simulink model "KinarmFlankerTask_260119"  (R2019b)
settings: Solver=ode4  StartTime=0.0  StopTime=inf  FixedStep=BKIN_STEP_TIME  RelTol=1e-3  EnableMultiTasking=on
StartFcn:
  |  warndlg('Dexterit-E models cannot run under simulation. Please compile your model and run it from within Dexterit-E.');set_param(bdroot,'SimulationCommand','stop')
model workspace (MAT data in the model file):
  ANT_ON = 7
  BKIN_KINEMATIC_FRAME_SIZE = 400
  BKIN_STEP_TIME = 0.00025
  CENTRE_TARG_COL = 8
  CUE_DELAY = 12
  CUE_ON_TIME = 11
  CUE_RAND = 13
  CUE_TARG_COL = 9
  DISTRACT_TARG_COL = 7
  E_ARROWS_BOT = 19
  E_ARROWS_OFF = 23
  E_ARROWS_ON = 21
  E_ARROWS_TOP = 18
  E_CENTRE_LEFT = 14
  E_CENTRE_RIGHT = 15
  E_CONG = 16
  E_CORRECT = 22
  E_CUE_BOT = 7
  E_CUE_BOTH = 8
  E_CUE_CENT = 20
  E_CUE_NONE = 5
  E_CUE_OFF = 9
  E_CUE_TOP = 6
  E_DISTRACT_LEFT = 11
  E_DISTRACT_NEUT = 13
  E_DISTRACT_RIGHT = 12
  E_FALSE_START = 28
  E_INCONG = 17
  E_INCORRECT = 24
  E_LEFT_REACHED = 1
  E_NEUTRAL = 10
  E_NO_EVENT = 0
  E_RIGHT_REACHED = 2
  E_TIMED_OUT = 29
  E_TRIAL_END = 30
  E_TRIAL_START = 3
  E_WALLS_ON = 4
  FLICKER_ON = 9
  FLICKER_TIME = 10
  IMAGE_1 = 6
  IMAGE_2 = 7
  IMAGE_3 = 8
  LBARR_TARG_COL = 4
  LENGTH = 3
  LOAD_X = 1
  LOAD_Y = 2
  LWALL_TARG_COL = 3
  NEUT_ON = 8
  PERTURB_SET = 10
  POSTRESP_DELAY = 4
  RADIUS_VIS = 3
  RBARR_TARG_COL = 6
  REACH_DELAY = 1
  REACH_RAND = 2
  REACH_TO = 3
  RESULT_TARG_COL = 2
  RWALL_TARG_COL = 5
  SPRING_CONST = 5
  START_TARG_COL = 1
  STROKE_WIDTH = 11
  TARG_LENGTH = 3
  TARG_WIDTH = 4
  TEXT = 9
  TEXT_SIZE = 10
  WALL_SHAKE_TOGGLE = 6
  WIDTH = 4
  Width = 4
  X_LENGTH = 4
  Y_LENGTH = 5
  col_x = 1
  col_y = 2
undefined symbols (not defined in the file or in its folder): slselsubs
libraries: Video x10, General x3, KINARM_general x3, KINARM_EP_loads x2
settings Model: ModifiedComment=chris -- Wed Feb 16 09:18:30 2005 -- Version 1.1384  ModifiedHistory=Feb 16/05 - Add error repeat, add offset ramp  ExtModeArmWhenConnect=off  ExtModeLogAll=off  OrderedModelArguments=off  Creator=Chris Grebeldinger  LastModifiedBy=apark2
settings SolverCC: AutoInsertRateTranBlk=on
settings DataIOCC: SaveFormat=Array  SignalLoggingSaveFormat=ModelDataLogs  SaveOutput=off  SaveTime=off  ReturnWorkspaceOutputs=off  SignalLoggingName=sigsOut
settings OptimizationCC: BlockReduction=off  BooleanDataType=off  OptimizeBlockIOStorage=off  BufferReuse=off  GlobalBufferReuse=off  ExpressionFolding=off  ExpressionDepthLimit=2147483647  LocalBlockOutputs=off  InitFltsAndDblsToZero=on  LifeSpan=inf  OptimizeDataStoreBuffers=off  BusAssignmentInplaceUpdate=off
settings DebuggingCC: SaveWithParameterizedLinksMsg=none  UnderspecifiedInitializationDetection=Classic  MergeDetectMultiDrivingBlocksExec=none  SignalResolutionControl=TryResolveAllWithWarning  MultiTaskDSMMsg=warning  FcnCallInpInsideContextMsg=warning  BusObjectLabelMismatch=none  StateNameClashWarn=warning  StrictBusMsg=ErrorOnBusTreatedAsVector  SFUnexpectedBacktrackingDiag=warning  SFNoUnconditionalDefaultTransitionDiag=warning  SFExecutionAtInitializationDiag=none  ArithmeticOperatorsInVariantConditions=warning
settings HardwareCC: ProdBitPerPointer=32  ProdBitPerSizeT=32  ProdBitPerPtrDiffT=32  ProdLargestAtomicFloat=None  ProdWordSize=32  ProdLongLongMode=on  ProdHWDeviceType=Generic->32-bit x86 compatible  TargetLongLongMode=on  TargetIntDivRoundTo=Zero  TargetEndianess=LittleEndian  TargetHWDeviceType=Generic->32-bit x86 compatible
settings ModelReferenceCC: PropagateSignalLabelsOutOfModel=off
settings SFSimCC: SimCustomHeaderCode="#include \"stdlib.h\""  SimUseLocalCustomCode=off  SimParseCustomCode=off  CustomCodeUndefinedFunction=UseInterfaceOnly
settings RTWCC: Description=Simulink Real-Time  SystemTargetFile=slrt.tlc  TemplateMakefile=slrt_default_tmf  RTWUseLocalCustomCode=off  CustomSourceCode="#include \"stdlib.h\""  CodeExecutionProfiling=on
settings CodeAppCC: MaxIdLength=63  StateflowObjectComments=on
settings SimulinkRealTimeCC: TargetFcnLib=ansi_tfl_tmw.mat  GeneratePreprocessorConditionals=Disable all  PreserveStateflowLocalDataDimensions=off
settings ConfigComp: CovMetricSettings=dw  CovHtmlReporting=on  CovSaveCumulativeToWorkspaceVar=on  CovSaveSingleToWorkspaceVar=on  CovExternalEMLEnable=off

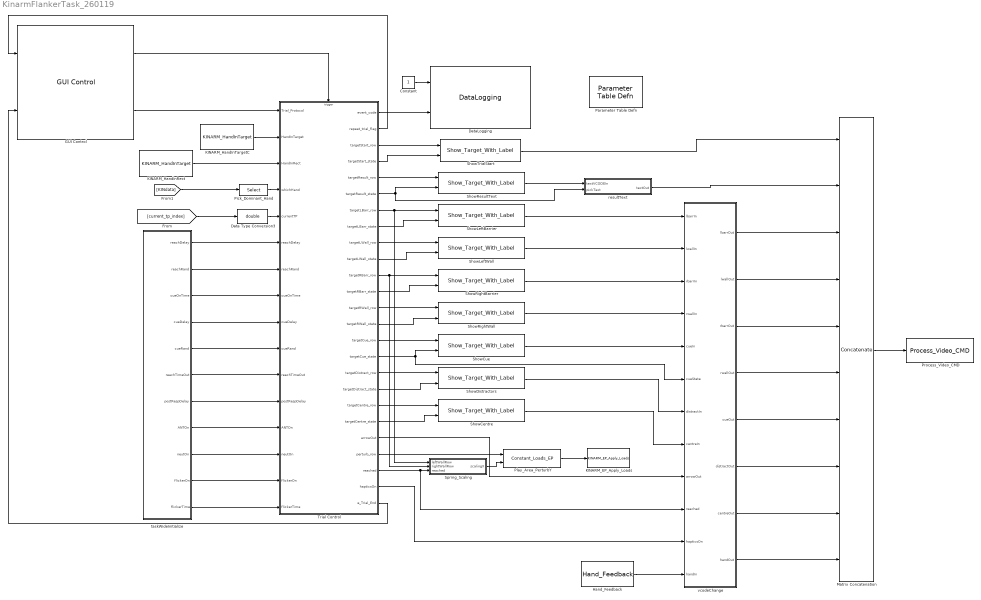
== system KinarmFlankerTask_260119 ==
  Constant : Constant
  Data Type Conversion3 : DataTypeConversion  OutDataTypeStr=double
  DataLogging : General/DataLogging  log_event_codes=on  log_analog_inputs=off  show_time_remaining=off  ecat_include=on
  GUI Control : General/GUI Control  task_version=1.0  show_repeat_trial_flag=on  use_custom_tp=off  target_type_str=Circle  Target_Type=1  XYcols=[1 2]  Vcols=3  Lcols=4  indices_padding=[0 0 0 0;0 0 0 0]  target_table_rows=64  load_table_rows=20  tp_table_rows=100
  Hand_Feedback : KINARM_general/Hand_Feedback  feedback_cntl_src=none
  KINARM_EP_Apply_Loads : KINARM_EP_loads/KINARM_EP_Apply_Loads  up_duration=1500  down_duration=1500  max_force=20
  KINARM_HandInRect : KINARM_general/KINARM_HandInTarget  use_dominant_hand=on  target_type=Rectangle  num_states=1  attribcol1=[X_LENGTH Y_LENGTH 0]  attribcol2=[0 0 0]  attribcol3=[0 0 0]  attribcol4=[0 0 0]  attribcol5=[0 0 0]
  KINARM_HandInTargetC : KINARM_general/KINARM_HandInTarget  use_dominant_hand=on  target_type=Circle  num_states=1  attribcol1=[RADIUS_VIS]  attribcol2=[0]  attribcol3=[0]  attribcol4=[0]  attribcol5=[0]
  Matrix Concatenation : Concatenate  NumInputs=10  Mode=Multidimensional array
  Parameter Table Defn : General/Parameter Table Defn  ShowInLibBrowser=0
  Pick_Dominant_Hand : Selector  NumberOfDimensions=2  InputPortWidth=3  IndexOptions=Index vector (dialog),Index vector (dialog)  Indices=[3],[1]  OutputSizes=slselsubs([(-2),(-2)],1),slselsubs([(-2),(-2)],2)
  Play_Area_PerturbY : KINARM_EP_loads/Constant_Loads_EP  use_dom_hand=on  loadcol=[LOAD_X LOAD_Y]  source=port  scaling=1  use_LH_coord=on
  Process_Video_CMD : Video/Process_Video_CMD  video_delay=50
  ShowCentre : Video/Show_Target_With_Label  target_type=Rectangle  num_states=2  attribcol1=[IMAGE_1 0 0 X_LENGTH Y_LENGTH 0 0 0 0]  attribcol2=[IMAGE_2 0 0 X_LENGTH Y_LENGTH 0 0 0 0]  attribcol3=[0 0 0 0 0 0 0 0 0]  attribcol4=[0 0 0 0 0 0 0 0 0]  attribcol5=[0 0 0 0 0 0 0 0 0]  stateindices_padding=[0 0;0 0;0 0;0 0;0 0]  source=dialog  opacity=100  target_display=Both subject and operator displays
  ShowCue : Video/Show_Target_With_Label  target_type=Rectangle  num_states=4  attribcol1=[0 0 0 0 0 0 TEXT IMAGE_1 TEXT_SIZE]  attribcol2=[0 0 0 0 0 0 TEXT IMAGE_1 TEXT_SIZE]  attribcol3=[0 0 0 0 0 0 TEXT IMAGE_1 TEXT_SIZE]  attribcol4=[0 0 0 0 0 0 TEXT IMAGE_1 TEXT_SIZE]  attribcol5=[0 0 0 0 0 0 0 0 0]  stateindices_padding=[0 0;0 0;0 0;0 0;0 0]  source=dialog  opacity=100  target_display=Both subject and operator displays
  ShowDistractors : Video/Show_Target_With_Label  target_type=Rectangle  num_states=3  attribcol1=[IMAGE_1 0 0 X_LENGTH Y_LENGTH 0 0 0 0]  attribcol2=[IMAGE_2 0 0 X_LENGTH Y_LENGTH 0 0 0 0]  attribcol3=[IMAGE_3 0 0 X_LENGTH Y_LENGTH 0 0 0 0]  attribcol4=[0 0 0 0 0 0 0 0 0]  attribcol5=[0 0 0 0 0 0 0 0 0]  stateindices_padding=[0 0;0 0;0 0;0 0;0 0]  source=dialog  opacity=100  target_display=Both subject and operator displays
  ShowLeftBarrier : Video/Show_Target_With_Label  target_type=Rectangle  num_states=1  attribcol1=[IMAGE_1 0 0 X_LENGTH Y_LENGTH 0 0 0 0]  attribcol2=[0 0 0 0 0 0 0 0 0]  attribcol3=[0 0 0 0 0 0 0 0 0]  attribcol4=[0 0 0 0 0 0 0 0 0]  attribcol5=[0 0 0 0 0 0 0 0 0]  stateindices_padding=[0 0;0 0;0 0;0 0;0 0]  source=dialog  opacity=100  target_display=Both subject and operator displays
  ShowLeftWall : Video/Show_Target_With_Label  target_type=Rectangle  num_states=2  attribcol1=[IMAGE_1 0 0 X_LENGTH Y_LENGTH 0 0 0 0]  attribcol2=[IMAGE_1 0 0 X_LENGTH Y_LENGTH 0 0 0 0]  attribcol3=[0 0 0 0 0 0 0 0 0]  attribcol4=[0 0 0 0 0 0 0 0 0]  attribcol5=[0 0 0 0 0 0 0 0 0]  stateindices_padding=[0 0;0 0;0 0;0 0;0 0]  source=dialog  opacity=100  target_display=Both subject and operator displays
  ShowResultText : Video/Show_Target_With_Label  target_type=Circle  num_states=4  attribcol1=[0 0 0 0 TEXT IMAGE_2 TEXT_SIZE]  attribcol2=[0 0 0 0 TEXT IMAGE_1 TEXT_SIZE]  attribcol3=[0 0 0 0 TEXT IMAGE_1 TEXT_SIZE]  attribcol4=[0 0 0 0 TEXT IMAGE_1 TEXT_SIZE]  attribcol5=[0 0 0 0 0 0 0]  stateindices_padding=[0 0 0 0;0 0 0 0;0 0 0 0;0 0 0 0;0 0 0 0]  source=dialog  opacity=100  target_display=Both subject and operator displays
  ShowRightBarrier : Video/Show_Target_With_Label  target_type=Rectangle  num_states=1  attribcol1=[IMAGE_1 0 0 X_LENGTH Y_LENGTH 0 0 0 0]  attribcol2=[0 0 0 0 0 0 0 0 0]  attribcol3=[0 0 0 0 0 0 0 0 0]  attribcol4=[0 0 0 0 0 0 0 0 0]  attribcol5=[0 0 0 0 0 0 0 0 0]  stateindices_padding=[0 0;0 0;0 0;0 0;0 0]  source=dialog  opacity=100  target_display=Both subject and operator displays
  ShowRightWall : Video/Show_Target_With_Label  target_type=Rectangle  num_states=2  attribcol1=[IMAGE_1 0 0 X_LENGTH Y_LENGTH 0 0 0 0]  attribcol2=[IMAGE_2 0 0 X_LENGTH Y_LENGTH 0 0 0 0]  attribcol3=[0 0 0 0 0 0 0 0 0]  attribcol4=[0 0 0 0 0 0 0 0 0]  attribcol5=[0 0 0 0 0 0 0 0 0]  stateindices_padding=[0 0;0 0;0 0;0 0;0 0]  source=dialog  opacity=100  target_display=Both subject and operator displays
  ShowTrialStart : Video/Show_Target_With_Label  target_type=Circle  num_states=1  attribcol1=[IMAGE_1 IMAGE_2 STROKE_WIDTH RADIUS_VIS 0 0 0]  attribcol2=[0 0 0 0 0 0 0]  attribcol3=[0 0 0 0 0 0 0]  attribcol4=[0 0 0 0 0 0 0]  attribcol5=[0 0 0 0 0 0 0]  stateindices_padding=[0 0 0 0;0 0 0 0;0 0 0 0;0 0 0 0;0 0 0 0]  source=dialog  opacity=100  target_display=Both subject and operator displays
  Spring_Scaling : Subsystem
  Trial Control : Stateflow chart  TreatAsAtomicUnit=on
  resultText : Subsystem
  taskWideInitialize : Subsystem
  vcodeChange : Subsystem
  wires:
  Trial Control/25(e_Trial_End) -> GUI Control/2
  Matrix Concatenation/1 -> Process_Video_CMD/1
  Trial Control/1(event_code) -> DataLogging/2
  Constant/1 -> DataLogging/1
  GUI Control/2 -> Trial Control/1(Trial_Protocol)
  Trial Control/2(repeat_trial_flag) -> GUI Control/1
  [current_tp_index] -> Data Type Conversion3/1
  ShowResultText/1 -> resultText/1(textVCODEIn)
  KINARM_HandInTargetC/1 -> Trial Control/2(HandInTarget)
  GUI Control/1 -> Trial Control/Trigger
  Data Type Conversion3/1 -> Trial Control/5(currentTP)
  Trial Control/18(targetDistract_state) -> ShowDistractors/2
  Trial Control/17(targetDistract_row) -> ShowDistractors/1
  Trial Control/13(targetRWall_row) -> ShowRightWall/1
  Trial Control/9(targetLWall_row) -> ShowLeftWall/1
  Trial Control/10(targetLWall_state) -> ShowLeftWall/2
  Trial Control/5(targetResult_row) -> ShowResultText/1
  Trial Control/6(targetResult_state) -> resultText/2(pickText), ShowResultText/2
  Trial Control/19(targetCentre_row) -> ShowCentre/1
  Trial Control/20(targetCentre_state) -> ShowCentre/2
  taskWideInitialize/1(reachDelay) -> Trial Control/6(reachDelay)
  taskWideInitialize/7(postRespDelay) -> Trial Control/12(postRespDelay)
  Trial Control/14(targetRWall_state) -> ShowRightWall/2
  resultText/1(textOut) -> Matrix Concatenation/2
  Play_Area_PerturbY/1 -> KINARM_EP_Apply_Loads/1
  Trial Control/24(hapticsOn) -> vcodeChange/11(hapticsOn)
  Trial Control/22(perturb_row) -> Play_Area_PerturbY/1
  Trial Control/3(targetStart_row) -> ShowTrialStart/1
  Trial Control/4(targetStart_state) -> ShowTrialStart/2
  ShowTrialStart/1 -> Matrix Concatenation/1
  taskWideInitialize/6(reachTimeOut) -> Trial Control/11(reachTimeOut)
  Trial Control/23(reached) -> Spring_Scaling/3(reached), vcodeChange/10(reached)
  ShowLeftWall/1 -> vcodeChange/2(lwallIn)
  ShowRightWall/1 -> vcodeChange/4(rwallIn)
  vcodeChange/6("distractOut ") -> Matrix Concatenation/8
  vcodeChange/7(centreOut) -> Matrix Concatenation/9
  Hand_Feedback/1 -> vcodeChange/12(handIn)
  ShowDistractors/1 -> vcodeChange/7(distractIn)
  ShowCentre/1 -> vcodeChange/8(centreIn)
  vcodeChange/2(lwallOut) -> Matrix Concatenation/4
  vcodeChange/4(rwallOut) -> Matrix Concatenation/6
  KINARM_HandInRect/1 -> Trial Control/3(HandInRect)
  Trial Control/21(arrowOut) -> vcodeChange/9(arrowOut)
  taskWideInitialize/8(ANTOn) -> Trial Control/13(ANTOn)
  Trial Control/15(targetCue_row) -> ShowCue/1
  Trial Control/16(targetCue_state) -> vcodeChange/6(cueState), ShowCue/2
  ShowCue/1 -> vcodeChange/5(cueIn)
  vcodeChange/5(cueOut) -> Matrix Concatenation/7
  vcodeChange/8(handOut) -> Matrix Concatenation/10
  Spring_Scaling/1(scalingX) -> Play_Area_PerturbY/2
  [KINdata] -> Pick_Dominant_Hand/1
  Pick_Dominant_Hand/1 -> Trial Control/4(whichHand)
  Trial Control/7(targetLBarr_row) -> ShowLeftBarrier/1, Spring_Scaling/1(leftWallRow)
  Trial Control/8(targetLBarr_state) -> ShowLeftBarrier/2
  ShowLeftBarrier/1 -> vcodeChange/1(lbarrIn)
  Trial Control/11(targetRBarr_row) -> ShowRightBarrier/1, Spring_Scaling/2(rightWallRow)
  Trial Control/12(targetRBarr_state) -> ShowRightBarrier/2
  ShowRightBarrier/1 -> vcodeChange/3(rbarrIn)
  vcodeChange/1(lbarrOut) -> Matrix Concatenation/3
  vcodeChange/3(rbarrOut) -> Matrix Concatenation/5
  taskWideInitialize/9(neutOn) -> Trial Control/14(neutOn)
  taskWideInitialize/2(reachRand) -> Trial Control/7(reachRand)
  taskWideInitialize/4(cueDelay) -> Trial Control/9(cueDelay)
  taskWideInitialize/5(cueRand) -> Trial Control/10(cueRand)
  taskWideInitialize/10(flickerOn) -> Trial Control/15(flickerOn)
  taskWideInitialize/11(flickerTime) -> Trial Control/16(flickerTime)
  taskWideInitialize/3(cueOnTime) -> Trial Control/8(cueOnTime)

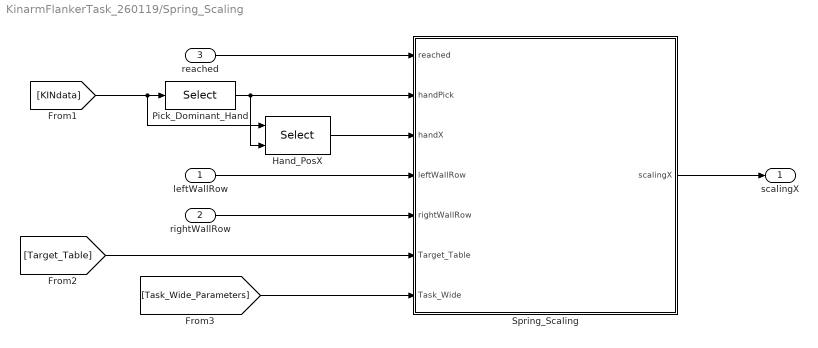
== system KinarmFlankerTask_260119/Spring_Scaling ==
  leftWallRow : Inport
  rightWallRow : Inport  Port=2
  reached : Inport  Port=3
  Hand_PosX : Selector  NumberOfDimensions=2  InputPortWidth=3  IndexOptions=Index vector (port),Index vector (dialog)  Indices=[3],[23]  OutputSizes=slselsubs([(-2),(-2)],1),slselsubs([(-2),(-2)],2)
  Pick_Dominant_Hand : Selector  NumberOfDimensions=2  InputPortWidth=3  IndexOptions=Index vector (dialog),Index vector (dialog)  Indices=[3],[1]  OutputSizes=slselsubs([(-2),(-2)],1),slselsubs([(-2),(-2)],2)
  Spring_Scaling : MATLAB Function  TreatAsAtomicUnit=on
  scalingX : Outport  VectorParamsAs1DForOutWhenUnconnected=off
  wires:
  Spring_Scaling/1(scalingX) -> scalingX/1
  reached/1 -> Spring_Scaling/1(reached)
  [Target_Table] -> Spring_Scaling/6(Target_Table)
  [KINdata] -> Hand_PosX/1, Pick_Dominant_Hand/1
  Pick_Dominant_Hand/1 -> Hand_PosX/2, Spring_Scaling/2(handPick)
  Hand_PosX/1 -> Spring_Scaling/3(handX)
  [Task_Wide_Parameters] -> Spring_Scaling/7(Task_Wide)
  leftWallRow/1 -> Spring_Scaling/4(leftWallRow)
  rightWallRow/1 -> Spring_Scaling/5(rightWallRow)

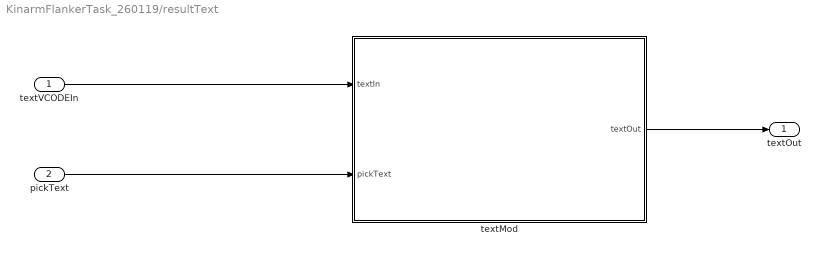
== system KinarmFlankerTask_260119/resultText ==
  textVCODEIn : Inport
  pickText : Inport  Port=2
  textMod : MATLAB Function  TreatAsAtomicUnit=on
  textOut : Outport
  wires:
  textMod/1(textOut) -> textOut/1
  textVCODEIn/1 -> textMod/1(textIn)
  pickText/1 -> textMod/2(pickText)

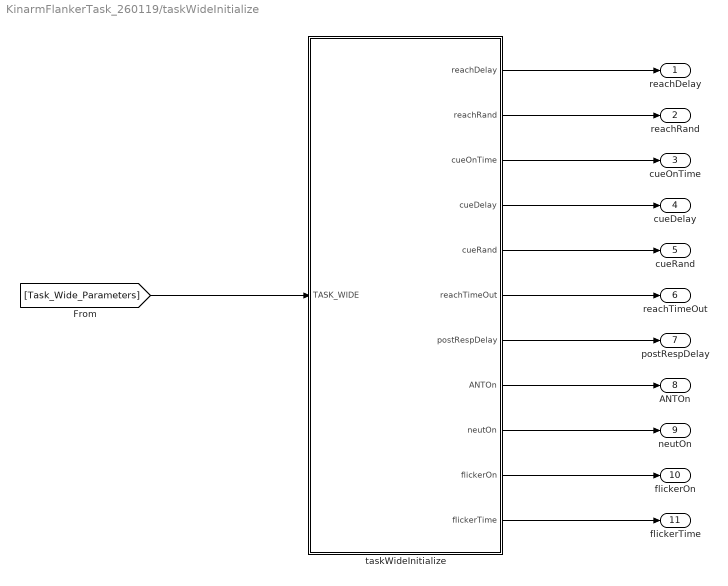
== system KinarmFlankerTask_260119/taskWideInitialize ==
  taskWideInitialize : MATLAB Function  TreatAsAtomicUnit=on
  reachDelay : Outport
  reachRand : Outport  Port=2
  cueOnTime : Outport  Port=3
  cueDelay : Outport  Port=4
  cueRand : Outport  Port=5
  reachTimeOut : Outport  Port=6
  postRespDelay : Outport  Port=7
  ANTOn : Outport  Port=8
  neutOn : Outport  Port=9
  flickerOn : Outport  Port=10
  flickerTime : Outport  Port=11
  wires:
  [Task_Wide_Parameters] -> taskWideInitialize/1(TASK_WIDE)
  taskWideInitialize/1(reachDelay) -> reachDelay/1
  taskWideInitialize/6(reachTimeOut) -> reachTimeOut/1
  taskWideInitialize/7(postRespDelay) -> postRespDelay/1
  taskWideInitialize/8(ANTOn) -> ANTOn/1
  taskWideInitialize/9(neutOn) -> neutOn/1
  taskWideInitialize/2(reachRand) -> reachRand/1
  taskWideInitialize/5(cueRand) -> cueRand/1
  taskWideInitialize/4(cueDelay) -> cueDelay/1
  taskWideInitialize/3(cueOnTime) -> cueOnTime/1
  taskWideInitialize/10(flickerOn) -> flickerOn/1
  taskWideInitialize/11(flickerTime) -> flickerTime/1

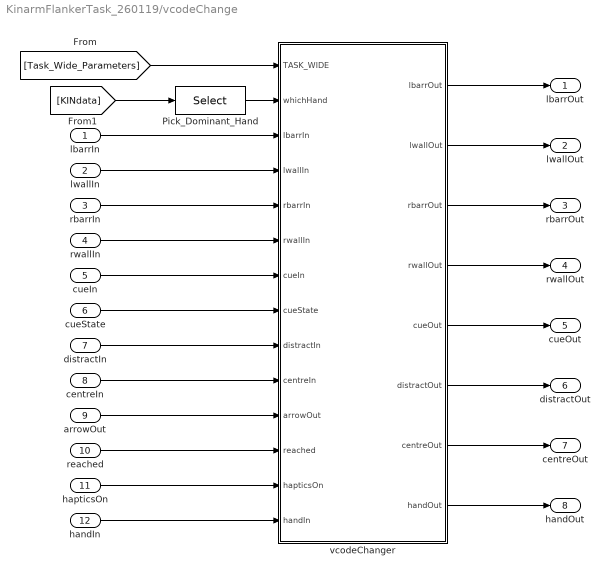
== system KinarmFlankerTask_260119/vcodeChange ==
  lbarrIn : Inport
  lwallIn : Inport  Port=2
  rbarrIn : Inport  Port=3
  rwallIn : Inport  Port=4
  cueIn : Inport  Port=5
  cueState : Inport  Port=6
  distractIn : Inport  Port=7
  centreIn : Inport  Port=8
  arrowOut : Inport  Port=9
  reached : Inport  Port=10
  hapticsOn : Inport  Port=11
  handIn : Inport  Port=12
  Pick_Dominant_Hand : Selector  NumberOfDimensions=2  InputPortWidth=3  IndexOptions=Index vector (dialog),Index vector (dialog)  Indices=[3],[1]  OutputSizes=slselsubs([(-2),(-2)],1),slselsubs([(-2),(-2)],2)
  "vcodeChanger " : MATLAB Function  TreatAsAtomicUnit=on
  lbarrOut : Outport
  lwallOut : Outport  Port=2
  rbarrOut : Outport  Port=3
  rwallOut : Outport  Port=4
  cueOut : Outport  Port=5
  "distractOut " : Outport  Port=6
  centreOut : Outport  Port=7
  handOut : Outport  Port=8
  wires:
  hapticsOn/1 -> "vcodeChanger "/13(hapticsOn)
  "vcodeChanger "/7(centreOut) -> centreOut/1
  centreIn/1 -> "vcodeChanger "/10(centreIn)
  reached/1 -> "vcodeChanger "/12(reached)
  [Task_Wide_Parameters] -> "vcodeChanger "/1(TASK_WIDE)
  "vcodeChanger "/6(distractOut) -> "distractOut "/1
  distractIn/1 -> "vcodeChanger "/9(distractIn)
  lwallIn/1 -> "vcodeChanger "/4(lwallIn)
  rwallIn/1 -> "vcodeChanger "/6(rwallIn)
  "vcodeChanger "/2(lwallOut) -> lwallOut/1
  "vcodeChanger "/4(rwallOut) -> rwallOut/1
  arrowOut/1 -> "vcodeChanger "/11(arrowOut)
  cueIn/1 -> "vcodeChanger "/7(cueIn)
  "vcodeChanger "/5(cueOut) -> cueOut/1
  cueState/1 -> "vcodeChanger "/8(cueState)
  handIn/1 -> "vcodeChanger "/14(handIn)
  "vcodeChanger "/8(handOut) -> handOut/1
  [KINdata] -> Pick_Dominant_Hand/1
  Pick_Dominant_Hand/1 -> "vcodeChanger "/2(whichHand)
  rbarrIn/1 -> "vcodeChanger "/5(rbarrIn)
  lbarrIn/1 -> "vcodeChanger "/3(lbarrIn)
  "vcodeChanger "/1(lbarrOut) -> lbarrOut/1
  "vcodeChanger "/3(rbarrOut) -> rbarrOut/1

== matlab function KinarmFlankerTask_260119/vcodeChange/vcodeChanger  ==
  data: lbarrOut output; lwallOut output; rbarrOut output; rwallOut output; cueOut output; distractOut output; centreOut output; TASK_WIDE input; whichHand input; lbarrIn input; lwallIn input; rbarrIn input; rwallIn input; cueIn input; cueState input; distractIn input; centreIn input; arrowOut input; reached input; hapticsOn input; POSTRESP_DELAY parameter; BKIN_STEP_TIME parameter; handIn input; handOut output; WALL_SHAKE_TOGGLE parameter
function [lbarrOut, lwallOut, rbarrOut, rwallOut, cueOut, distractOut, centreOut, handOut] =...
    fcn(TASK_WIDE, whichHand, lbarrIn, lwallIn, rbarrIn, rwallIn, cueIn, cueState, distractIn, centreIn, arrowOut, reached, hapticsOn, POSTRESP_DELAY, BKIN_STEP_TIME, handIn, WALL_SHAKE_TOGGLE)
%this function modifies the centre arrow and wall movement (if reached correctly)
%stroop vcode is routed through this function just for cleaner simulink

%initialize taskwides
postReachDelay = TASK_WIDE(POSTRESP_DELAY); %time after reach completed
shakeOnOff = TASK_WIDE(WALL_SHAKE_TOGGLE); %turn on or off the visual shaking of the walls
dt = BKIN_STEP_TIME;
speedScalar = 1000/postReachDelay;
shakeScalar = 1/8; %speed of wall shake
shakeLim = 0.01; %distance of shaking

%set output vcodes
lbarrOut = lbarrIn;
lwallOut = lwallIn;
rbarrOut = rbarrIn;
rwallOut = rwallIn;
if (whichHand == 2) %flip barriers and walls for other hand
    lbarrOut = rbarrIn;
    lwallOut = rwallIn;
    rbarrOut = lbarrIn;
    rwallOut = lwallIn;
end
centreOut = centreIn;
distractOut = zeros(4,70); %make four distractor arrows
distractOut(1,:) = distractIn; %far left arrow
distractOut(1,3) = distractIn(1,3)-2*distractIn(1,10); %shift far left arrow to correct position
distractOut(2,:) = distractIn; %left arrow
distractOut(2,3) = distractIn(1,3)-distractIn(1,10); %shift left arrow to correct position
distractOut(3,:) = distractIn; %right arrow
distractOut(3,3) = distractIn(1,3)+distractIn(1,10); %shift right arrow to correct position
distractOut(4,:) = distractIn; %far right arrow
distractOut(4,3) = distractIn(1,3)+2*distractIn(1,10); %shift far right arrow to correct position
    
cueOut = zeros(2,70); %make 2 cue targets
cueOut(1,:) = cueIn; %top/centre cue target
cueOut(2,:) = cueIn; %bottom cue target
handOut = handIn; 

%get arrow vcodes
if (arrowOut == 2) %arrows below the start target
    distractOut(1:4,4) = distractIn(1:4,4) - 2*(distractIn(1:4,4) - lwallOut(1,4)); %shift distractor arrows below the start target
    centreOut(1,4) = distractIn(1,4) - 2*(distractIn(1,4) - lwallOut(1,4)); %shift centre arrows below the start target
end

%show different cues
if (cueState == 1) %show cue above start target
    cueOut(1,4) = cueIn(1,4); %top cue on
    cueOut(2,2) = 0; %turn off bottom cue
elseif (cueState == 2) %cue below the start target
    cueOut(1,2) = 0; %top cue off
    cueOut(2,4) = cueIn(1,4) - 2*(distractIn(1,4) - lwallOut(1,4)); %bottom cue on
elseif (cueState == 3) %both cues on
    cueOut(1,4) = cueIn(1,4); %top cue on
    cueOut(2,4) = cueIn(1,4) - 2*(distractIn(1,4) - lwallOut(1,4)); %bottom cue on
end
if (cueState == 4) %show centre cue by changing the cursor to the cue
    handOut(1,2) = 0; %turn hands off
    handOut(2,2) = 0; %turn hands off
    cueOut(1,4) = cueIn(1,4) - (distractIn(1,4) - lwallOut(1,4)) - 0.002; %show top cue in centre position (0.2cm adjustment otherwise it looks weird as the astrisk is a text in superscript)
    cueOut(2,2) = 0; %turn off second cue
end

%set up centre arrow movement
persistent atTime0 moveDistX shakeWall
if (isempty(atTime0))
    atTime0 = 0;
    moveDistX = 0;
    shakeWall = 0;
end

if (hapticsOn == 1) %if reached successfully
    if (reached == 1) %if left wall reached
        if (shakeWall <= shakeLim && shakeOnOff == 1) %if wallshake is on
            shakeWall = shakeWall + dt*shakeScalar; %increase shake
        else
            shakeWall = 0;
        end
        lwallOut(1,3) = lwallOut(1,3)-shakeWall; %left wall shake
        moveDistX = moveDistX + dt*(centreIn(1,3)-distractOut(1,3))*speedScalar; %move centre arrow left
        centreOut(1,3) = centreOut(1,3)-moveDistX; %centre arrow shift
    elseif (reached == 2) %if right wall reached
        if (shakeWall <= shakeLim && shakeOnOff == 1)
            shakeWall = shakeWall + dt*shakeScalar; %increase shake
        else
            shakeWall = 0;
        end
        rwallOut(1,3) = rwallOut(1,3)+shakeWall;
        moveDistX = moveDistX + dt*(centreIn(1,3)-distractOut(4,3))*speedScalar; %move centre arrow right
        centreOut(1,3) = centreOut(1,3)-moveDistX;
    end
end

if (reached == 0) %reset the wallshake movement
    atTime0 = [];
end

== stateflow chart KinarmFlankerTask_260119/Trial Control ==
  state Initialize/
    %setup the variables
    targetStart_row = Trial_Protocol(START_TARG_COL); %target to start the trials
    targetResult_row = Trial_Protocol(RESULT_TARG_COL); %result target
    targetLBarr_row = Trial_Protocol(LBARR_TARG_COL); %left barrier
    targetLWall_row = Trial_Protocol(LWALL_TARG_COL); %show left virtual wall
    targetRBarr_row = Trial_Protocol(RBARR_TARG_COL); %right barrier
    targetRWall_row = Trial_Protocol(RWALL_TARG_COL); %show right virtual wall
    targetDistract_row = Trial_Protocol(DISTRACT_TARG_COL); %show distractor arrows
    targetCentre_row = Trial_Protocol(CENTRE_TARG_COL); %show centre arrows
    targetCue_row = Trial_Protocol(CUE_TARG_COL); %show cue target
    targetStart_state = 0; %turn off start target
    targetResult_state = 0; %turn off result target
    targetLBarr_state = 0; %turn off left barrier
    targetLWall_state = 0; %turn off left virtual wall
    targetRBarr_state = 0; %turn off right barrier
    targetRWall_state = 0; %turn off right virtual wall
    targetDistract_state = 0; %turn off distractor arrows
    targetCentre_state = 0; %turn off centre target
    targetCue_state = 0; %turn off cue target
    hapticsOn = 0; %no haptic feedback
    reached = 0; %outputs the wall reached flag (1 = left, 2 = right)
  state MainTrial
    state startTrial/
      %get the Distractor and Centre arrow directions, Cue position, arrow position
      %cue position and arrow position irrelevant for baseFlanker task
      entry:
      targetStart_state = 1; %turn on Start Target
      perturb_row = Trial_Protocol(PERTURB_SET); %get the perturbation row
      [distrState,centreState,cueOut,arrowOut] = pickFlank(currentTP,ANTOn,neutOn); %get flanker stuff
      targetResult_state = 0; %turn off result text
      randReach = reachRand*rand(); %get a random reach time
      randCue = cueRand*rand(); %get a random cue/fixation time
      event_code = E_TRIAL_START;
    state showInstruction/
      %show start targ
      targetStart_state = 1;
      targetResult_state =1;
    state checkForHandOut/
      %get the event codes for the Cue Target
      state wallsOn/
        %turn Walls on
        event_code = E_WALLS_ON;
        targetStart_state = 1;
        targetLBarr_state = 1;
        targetLWall_state = 1;
        targetRBarr_state = 1;
        targetRWall_state = 1;
        targetResult_state = 0;
      state cueOn/
        %display the Cue(s)
        targetCue_state = cueOut;
      state cueEvents/
        %cue event codes
        state noCue/
          event_code = E_CUE_NONE;
        state topCue/
          event_code = E_CUE_TOP;
        state bottomCue/
          event_code = E_CUE_BOT;
        state bothCue/
          event_code = E_CUE_BOTH;
        state centreCue/
          event_code = E_CUE_CENT;
      state cueIsOn/
        %display the Cue/fixation
        targetCue_state = 1;
        event_code = E_CUE_TOP;
      state cueOff/
        %turn off the Cues
        event_code = E_CUE_OFF;
        targetCue_state = 0;
      wallsOn -> (junction 690) [order 1] : %ANT version
          | [ANTOn == 1]
      (junction 690) -> cueOn : %time before cue turns on
          | after(randReach+reachDelay,msec)
      wallsOn -> (junction 692) [order 2] : %baseFlanker version
          | [ANTOn == 0]
      (junction 692) -> cueIsOn : %time before cue turns on
          | after(randReach+reachDelay,msec)
      cueOn -> centreCue [order 2] : [cueOut == 4]
      cueOn -> bothCue [order 5] : [cueOut == 3]
      cueOn -> bottomCue [order 4] : [cueOut == 2]
      cueOn -> topCue [order 1] : [cueOut == 1]
      cueOn -> noCue [order 3] : [cueOut == 0]
      cueIsOn -> cueOff : %time cue stays on
          | after(cueOnTime,msec)
      cueEvents -> cueOff : %time cue stays on
          | after(cueOnTime,msec)
    state falseStart/
      %left Start Target too early
      event_code = E_FALSE_START;
      targetResult_state = 4;
    state reset/
      %turn off result text
      targetResult_state = 0;
    state centreEvents/
      %event codes for centre arrow
      state centreLeft/
        event_code = E_CENTRE_LEFT;
      state centreRight/
        event_code = E_CENTRE_RIGHT;
    state distractEvents/
      %Distractor event codes
      state distractLeft/
        event_code = E_DISTRACT_LEFT;
      state distractRight/
        event_code = E_DISTRACT_RIGHT;
      state distractNeut/
        event_code = E_DISTRACT_NEUT;
    state nice3/
    state trialEvents/
      %event codes for trial type
      state neutral/
        event_code = E_NEUTRAL;
      state incong/
        event_code = E_INCONG;
      state cong/
        event_code = E_CONG;
    state nice1/
    state nice4/
    state flankAppear/
      %show Centre and Distractors
      targetDistract_state = distrState;
      targetCentre_state = centreState;
      flankDir = mod(currentTP,2);
      event_code = E_ARROWS_ON;
      targetStart_state = 0;
    state nice2/
    state arrowSide/
      %arrows position top or bottom
      state arrowsBot/
        event_code = E_ARROWS_BOT;
      state arrowsTop/
        event_code = E_ARROWS_TOP;
    state nice6/
    state leftReach/
      %left Wall reached
      event_code = E_LEFT_REACHED;
    state leftCorrect/
      %left reach correct
      reached = 1; %reached left wall
    state nice5/
    state rightCorrect/
      %right reach correct
      reached = 2; %reached right wall
    state rightReach/
      %right Wall reached
      event_code = E_RIGHT_REACHED;
    state flicker/
      %turn off arrows before trial is done
      targetDistract_state = 0;
      targetCentre_state = 0;
      event_code = E_ARROWS_OFF;
    state resultEvent/
      %send out result event
      state correct/
        %reach was correct and
        %turn on haptic feedback
        hapticsOn = 1;
        event_code = E_CORRECT;
      state timeoutTrial/
        %didnt reach a Wall
        event_code = E_TIMED_OUT;
        targetResult_state = 3;
        targetStart_state = 0;
      state incorrect/
        %reach was incorrect and show
        %text on screen
        event_code = E_INCORRECT;
        targetResult_state = 2;
    state trialEnd/
      %turn off all targets
      event_code = E_TRIAL_END;
      hapticsOn = 0;
      reached = 0;
      targetStart_state = 0;
      targetResult_state = 0;
      targetLBarr_state = 0;
      targetLWall_state = 0;
      targetRBarr_state = 0;
      targetRWall_state = 0;
      targetDistract_state = 0;
      targetCentre_state = 0;
      targetCue_state = 0;
    state leftWrong/
      %turn off wrong Wall
      targetRWall_state = 0;
    state rightWrong/
      %turn off wrong wall
      targetLWall_state = 0;
    showInstruction -> startTrial : %check hand in target
        | [HandInTarget(targetStart_row) == 1]
    checkForHandOut -> falseStart : %hand left the Start Target
        | [HandInTarget(targetStart_row) == 0]
    falseStart -> (junction 821) : %hand went back into start
        | [HandInTarget(targetStart_row) == 1]
    (junction 821) -> reset : after(postRespDelay/2,msec)
    startTrial -> reset
    reset -> wallsOn : %check hand in target
        | [HandInTarget(targetStart_row) == 1]
    nice3 -> distractLeft [order 3] : %Distractors left
        | [distrState == 1]
    nice2 -> centreLeft [order 2] : %Centre arrow points left
        | [centreState == 1]
    nice3 -> distractRight [order 2] : %Distractors right
        | [distrState == 2]
    centreEvents -> nice3 : after(1,msec)
    nice2 -> centreRight [order 1] : %Centre arrow points right
        | [centreState == 2]
    nice1 -> neutral [order 2] : %neutral (TP > 40 are neutral)
        | [currentTP > 40]
    nice3 -> distractNeut [order 1] : %neutral distractors
        | [distrState == 3]
    distractEvents -> nice4 : after(1,msec)
    nice1 -> incong [order 3] : %incongruent
    trialEvents -> nice2 : after(1,msec)
    nice1 -> cong [order 1] : %congruent (distractor+centre arrow states
        | %add up to an even number for congruent trials)
        | [currentTP < 41 &&...
        |  (mod(distrState+centreState,2) == 0)]
    flankAppear -> nice1 : after(1,msec)
    nice4 -> nice5 [order 1] : %baseFlanker
        | [ANTOn == 0]
    nice4 -> arrowsTop [order 3] : %arrows above cue
        | [arrowOut == 1]
    nice4 -> arrowsBot [order 2] : %arrows below cue
        | [arrowOut == 2]
    cueOff -> flankAppear : %time before arrows turn on
        | after(cueDelay+randCue,msec)
    arrowSide -> nice5 : after(1,msec)
    nice6 -> (junction 784) [order 2] : %right hand used
        | [whichHand == 1]
    (junction 784) -> leftReach [order 2] : %right hand in left Wall
        | [HandInRect(targetLBarr_row)==1]
    (junction 784) -> rightReach [order 1] : %right hand in right Wall
        | [HandInRect(targetRBarr_row)==1]
    leftReach -> leftCorrect [order 1] : %odd TP has Centre point left
        | [flankDir == 1]
    (junction 785) -> leftReach [order 1] : %left hand in left Wall
        | [HandInRect(targetRBarr_row)==1]
    leftReach -> (junction 801) [order 2] : after(1,msec)
    leftCorrect -> correct : after(1,msec)
    nice5 -> nice6 [order 2] : %No arrow flickers
        | [flickerOn == 0]
    nice5 -> (junction 810) [order 1] : %arrows flicker
        | [flickerOn == 1]
    rightReach -> rightCorrect [order 1] : %even TP has Centre point right
        | [flankDir == 0]
    rightCorrect -> correct : after(1,msec)
    (junction 810) -> flicker : after(flickerTime,msec)
    nice6 -> (junction 785) [order 3] : %left hand used
        | [whichHand == 2]
    (junction 785) -> rightReach [order 2] : %left hand in right wall
        | [HandInRect(targetLBarr_row)==1]
    rightReach -> (junction 798) [order 2] : after(1,msec)
    flicker -> nice6
    nice6 -> timeoutTrial [order 1] : %didnt reach in time
        | after(reachTimeOut,msec)
    (junction 798) -> leftWrong [order 1] : %right hand
        | [whichHand == 1]
    (junction 798) -> rightWrong [order 2] : %left hand
        | [whichHand == 2]
    (junction 801) -> leftWrong [order 2] : %left hand
        | [whichHand == 2]
    (junction 801) -> rightWrong [order 1] : %right hand
        | [whichHand == 1]
    leftWrong -> incorrect
    rightWrong -> incorrect
    resultEvent -> trialEnd : after(postRespDelay,msec)
  state Inter_Trial_State/
    %turn off all
    entry:
    event_code = 0;
    repeat_trial_flag = 0;
    hapticsOn = 0;
    reached = 0;
    targetStart_state = 0;
    targetResult_state = 0;
    targetLBarr_state = 0;
    targetLWall_state = 0;
    targetRBarr_state = 0;
    targetRWall_state = 0;
    targetDistract_state = 0;
    targetCentre_state = 0;
    targetCue_state = 0;
    e_Trial_End;
  state RepeatTrial/
    entry:
    repeat_trial_flag = 1;
  (default) -> Initialize
  Initialize -> showInstruction : %wait for task to start
      | [currentTP > 0]
  Inter_Trial_State -> startTrial : after(1,msec)
  RepeatTrial -> Inter_Trial_State : after(1,msec)
  MainTrial -> RepeatTrial : e_ExitTrialNow
      | % e_ExitTrialNow event occurs if the
      | % Dex pause is pressed by the operator
  trialEnd -> Inter_Trial_State : after(1,msec)
  data: stateDistr function_output; stateCentre function_output; nowTP function_input; outCue function_output; ANTIn function_input; outArrow function_output; neutIn function_input; event_code output [0..]; repeat_trial_flag output; targetStart_row output; targetStart_state output; Trial_Protocol input; HandInTarget input; HandInRect input; whichHand input; targetResult_row output; targetResult_state output; targetLBarr_row output; targetLBarr_state output; targetLWall_row output; targetLWall_state output; targetRBarr_row output; targetRBarr_state output; targetRWall_row output; targetRWall_state output; targetCue_row output; targetCue_state output; targetDistract_row output; targetDistract_state output; targetCentre_row output; targetCentre_state output; arrowOut output; perturb_row output; reached output; hapticsOn output; currentTP input; reachDelay input; reachRand input; cueOnTime input; cueDelay input; cueRand input; reachTimeOut input; postRespDelay input; textOut local; distrState local; centreState local; flankDir local; ANTOn input; cueOut local; neutOn input; flickerOn input; flickerTime input; randReach local; randCue local
  events: e_clk input RISING_EDGE_EVENT; e_ExitTrialNow input RISING_EDGE_EVENT; e_Trial_End output EITHER_EDGE_EVENT
  function [stateDistr,stateCentre,outCue,outArrow] = pickFlank(nowTP,ANTIn,neutIn):
    | function [stateDistr,stateCentre,outCue,outArrow] = pickFlank(nowTP,ANTIn,neutIn)
    | %This function sets up an array for picking the state of distractors and
    | %centre arrows (state dictates image which is left arrow = 1, right arrow = 2,
    | %neutral only for distractor = 3) also picks the cue type (0 = no cue, 
    | %1 = cue on top, 2 = cue on bottom, 3 = cue on top and bottom, 4 = cue centre) 
    | %and arrows position (1 = arrows on top, 2 = arrows on bottom) must have 
    | %60 TP for all types of trials to appear (distract(3)*arrow(2)*cue(5)*arrows(2) = 60)
    | 
    | %% set up array to pull distractor and centre arrow states
    | 
    | %50% congruent/incongruent array for stroop target colour-text pairs
    | flankerNeut = [1 2 2 1 1 2 2 1 1 2 2 1 1 2 2 1 1 2 2 1 1 2 2 1 1 2 2 1 1 2 2 1 3 3 3 3 3 3 3 3 3 3 3 3 3 3 3 3;... %state of distractor arrow (1 = left, 2 = right, 3 = neut)
    |                 1 2 1 2 1 2 1 2 1 2 1 2 1 2 1 2 1 2 1 2 1 2 1 2 1 2 1 2 1 2 1 2 1 2 1 2 1 2 1 2 1 2 1 2 1 2 1 2;... %state of centre arrow (1 = left, 2 = right)
    |                 0 0 0 0 1 1 1 1 3 3 3 3 0 0 0 0 2 2 2 2 3 3 3 3 4 4 4 4 4 4 4 4 4 4 4 4 0 0 1 1 0 0 2 2 3 3 3 3;... %0=cue off, 1=cue top, 2=cue bottom, 3=cue top and bottom, 4 = cue centre
    |                 1 1 1 1 1 1 1 1 1 1 1 1 2 2 2 2 2 2 2 2 2 2 2 2 1 1 1 1 2 2 2 2 1 1 2 2 1 1 1 1 2 2 2 2 1 1 2 2];   %arrows top = 1, arrows bottom = 2
    |             
    | flankerTight = [1 2 2 1 1 2 2 1 1 2 2 1 1 2 2 1 1 2 2 1 1 2 2 1 1 2 2 1 1 2 2 1;... %state of distractor arrow (1 = left, 2 = right)
    |                 1 2 1 2 1 2 1 2 1 2 1 2 1 2 1 2 1 2 1 2 1 2 1 2 1 2 1 2 1 2 1 2;... %state of centre arrow (1 = left, 2 = right)
    |                 0 0 0 0 1 1 1 1 3 3 3 3 0 0 0 0 2 2 2 2 3 3 3 3 4 4 4 4 4 4 4 4;... %0=cue off, 1=cue top, 2=cue bottom, 3=cue top and bottom, 4 = cue centre
    |                 1 1 1 1 1 1 1 1 1 1 1 1 2 2 2 2 2 2 2 2 2 2 2 2 1 1 1 1 2 2 2 2];   %arrows top = 1, arrows bottom = 2
    |             
    | %% output variables
    | 
    | if (neutIn == 1) %keep neutral trials
    |     flankerArray = flankerNeut; %groups of 48 trials in block table MUST
    | else %remove neutral trials if unwanted 
    |     flankerArray = flankerTight; %groups of 32 trials in block table MUST
    | end
    | 
    | %output the state of distractor and centre arrows for baseFlanker and ANT
    | stateDistr = flankerArray(1,nowTP); % pick distractor state 
    | stateCentre = flankerArray(2,nowTP); % pick centre state
    | if (ANTIn == 1) %if the ANT version is used
    |     outCue = flankerArray(3,nowTP);
    |     outArrow = flankerArray(4,nowTP);
    | else %if baseFlanker is used don't alter the cue or arrow positions
    |     outCue = 0;
    |     outArrow = 0;
    | end

== matlab function KinarmFlankerTask_260119/taskWideInitialize/taskWideInitialize ==
  data: TASK_WIDE input; reachDelay output; reachRand output; cueOnTime output; cueDelay output; cueRand output; reachTimeOut output; postRespDelay output; REACH_DELAY parameter; REACH_TO parameter; POSTRESP_DELAY parameter; ANTOn output; ANT_ON parameter; NEUT_ON parameter; neutOn output; REACH_RAND parameter; CUE_RAND parameter; CUE_DELAY parameter; flickerOn output; flickerTime output; FLICKER_ON parameter; FLICKER_TIME parameter; CUE_ON_TIME parameter
function [reachDelay, reachRand, cueOnTime, cueDelay, cueRand, reachTimeOut, postRespDelay, ANTOn, neutOn, flickerOn, flickerTime] =...
    fcn(TASK_WIDE, REACH_DELAY, REACH_TO, POSTRESP_DELAY, ANT_ON, NEUT_ON, REACH_RAND, CUE_RAND, CUE_DELAY, FLICKER_ON, FLICKER_TIME, CUE_ON_TIME)  

%% task wide parameter outputs
reachDelay = TASK_WIDE(REACH_DELAY); %time to hold hand in the Start Target to begin trials
reachRand = TASK_WIDE(REACH_RAND); %random added time to reachDelay
cueOnTime = TASK_WIDE(CUE_ON_TIME); %time the cue/fixation stays on
cueDelay = TASK_WIDE(CUE_DELAY); %time between cue/fixation turning off and arrows turning on
cueRand = TASK_WIDE(CUE_RAND); %random time added to cueDelay
reachTimeOut = TASK_WIDE(REACH_TO); %alloted time for reaching left or right before a Too slow! text
postRespDelay = TASK_WIDE(POSTRESP_DELAY); %time between trials
ANTOn = TASK_WIDE(ANT_ON); %turn on the attention network test on (1) or off (0)
neutOn = TASK_WIDE(NEUT_ON); %turn on (1) or off (0) the neutral trials (must use TP1-48 and each block must have groups of 48 trials)
flickerOn = TASK_WIDE(FLICKER_ON); %turn on or off the arrows turning on and off quickly (some studies have used this)
flickerTime = TASK_WIDE(FLICKER_TIME); %duration the arrows will stay on if flickerOn = 1

== matlab function KinarmFlankerTask_260119/Spring_Scaling/Spring_Scaling ==
  data: reached input; handPick input; handX input; leftWallRow input; rightWallRow input; Target_Table input; Task_Wide input; SPRING_CONST parameter; scalingX output; X_LENGTH parameter
function scalingX  = Spring_Scaling(reached, handPick, handX, leftWallRow, rightWallRow, Target_Table, Task_Wide, SPRING_CONST, X_LENGTH)
%Make the Barriers push the hand back

%initialize variables
springConst = Task_Wide(SPRING_CONST)* 10; %10 is a minor adjustment for cm -> m conversion (20 feels good)

if (handPick == 1) %if right hand used
    leftBarrier = Target_Table(leftWallRow,1)*0.01 + Target_Table(leftWallRow,X_LENGTH)*0.005; %centre of Barrier and half of the length is the right side of the left Barrier
    rightBarrier = Target_Table(rightWallRow,1)*0.01 - Target_Table(rightWallRow,X_LENGTH)*0.005;
else %if left hand used
    leftBarrier = Target_Table(rightWallRow,1)*0.01 + Target_Table(rightWallRow,X_LENGTH)*0.005; %swap left and right Barriers
    rightBarrier = Target_Table(leftWallRow,1)*0.01 - Target_Table(leftWallRow,X_LENGTH)*0.005;
end

%check if the hands are in the Barriers
leftCHECK = double(handX < leftBarrier); %check left Barrier
rightCHECK = double(handX > rightBarrier); %check right Barrier

%% SPRING SCALING 
% set conditions for the scaling to push the hand back into the centre
scalingX = 0;
if (reached == 1) %only start spring scaling once left Barrier is reached
    if (leftCHECK) %check left Barrier condition
        if (handPick == 1) %accounts for flipped left/right hand usage
            scalingX = springConst * (leftBarrier - handX); %scaling based on basic spring force equation f=kx (force = constant*distance)
            if (leftBarrier - handX > 10) %safety
                scalingX = springConst * 10;
            end
        else %flipped scaling to account for left/right hand usage
            scalingX = -springConst * (leftBarrier - handX);
            if (leftBarrier - handX > 10) %safety
                scalingX = -springConst * 10;
            end
        end
    else
        scalingX = 0;
    end
end

if (reached == 2) %hand reached right Barrier
    if (rightCHECK) %check right boundary condition
        if (handPick == 1) %left hand
            scalingX = -springConst * (rightBarrier - handX);
            if (handX - rightBarrier > 10) %safety
                scalingX = -springConst * 10;
            end
        else %right hand
            scalingX = springConst * (rightBarrier - handX);
            if (handX - rightBarrier > 10) %safety
                scalingX = springConst * 10;
            end
        end
    else
        scalingX = 0;
    end
end

== matlab function KinarmFlankerTask_260119/resultText/textMod ==
  data: textIn input; pickText input; textOut output
function textOut  = fcn(textIn, pickText)
%function modifies the trial result text with hardcoded text

textOut = textIn;
if (pickText == 1) %begin the task text
    str1 = ['Place your cursor in the circle to begin'];
elseif (pickText == 2) %incorrect trials output
    str1 = ['Incorrect!'];
elseif (pickText == 3) %timed out trials output
    str1 = ['Too slow!'];
elseif (pickText == 4) %false start trials output
    str1 = ['Stay inside!'];
else %checks errors
    str1 = ['Error'];
end
textOut(1,15:(length(str1)+14))=uint16(str1);  %str in letters
